simulink model "sfSupertransitionAPIExample"  (R2025b)
settings: Solver=VariableStepAuto  StartTime=0.0  StopTime=10.0  RelTol=1e-3
settings Model: Creator=The MathWorks, Inc.  LastModifiedBy=The MathWorks, Inc.
settings OptimizationCC: ReuseModelBlockBuffer=off
settings RTWCC: GPUComputeCapability=3.5

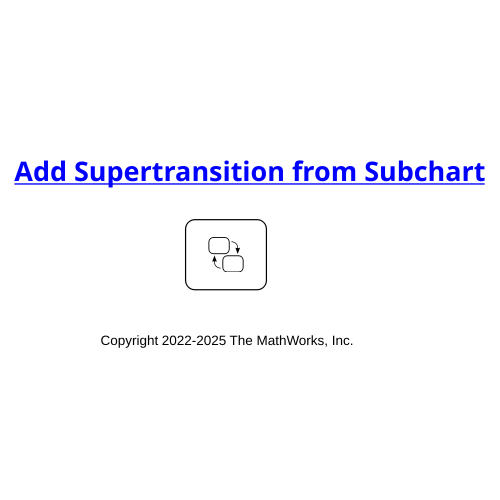
[thumbnail: Simulink's stored preview of the top-level diagram]
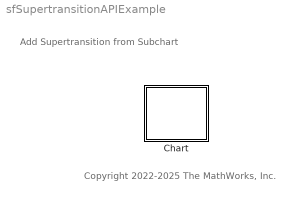
== system sfSupertransitionAPIExample ==
  note: Copyright 2022-2025 The MathWorks, Inc.
  note: Add Supertransition from Subchart
  Chart : Stateflow chart  TreatAsAtomicUnit=on

== stateflow chart sfSupertransitionAPIExample/Chart ==
  state A
